simulink model "HW5"  (R2023b)
settings: Solver=FixedStepAuto  StartTime=0.0  StopTime=100  FixedStep=0.01  RelTol=1e-3
settings Model: Creator=ArshiaGosh  LastModifiedBy=ArshiaGosh

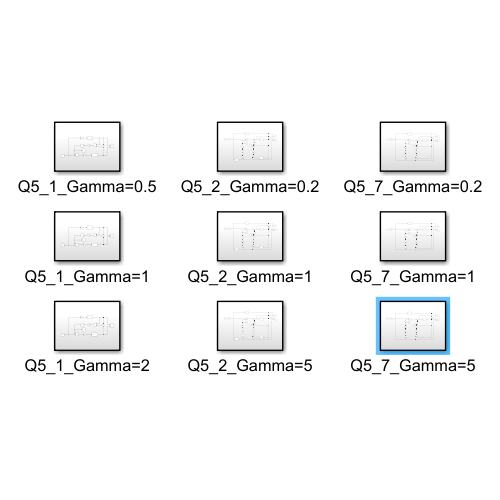
[thumbnail: Simulink's stored preview of the top-level diagram]
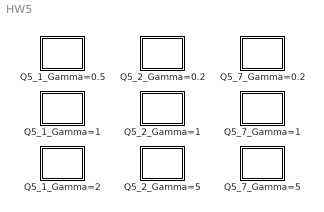
== system HW5 ==
  Q5_1_Gamma=0.5 : Subsystem
  Q5_1_Gamma=1 : Subsystem
  Q5_1_Gamma=2 : Subsystem
  Q5_2_Gamma=0.2 : Subsystem
  Q5_2_Gamma=1 : Subsystem
  Q5_2_Gamma=5 : Subsystem
  Q5_7_Gamma=0.2 : Subsystem
  Q5_7_Gamma=1 : Subsystem
  Q5_7_Gamma=5 : Subsystem

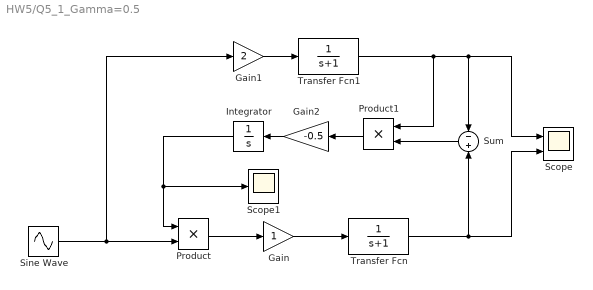
== system HW5/Q5_1_Gamma=0.5 ==
  Gain : Gain
  Gain1 : Gain  Gain=2
  Gain2 : Gain  Gain=-0.5
  Integrator : Integrator
  Product : Product
  Product1 : Product
  Scope : Scope  NumInputPorts=2
  Scope1 : Scope
  Sine Wave : Sin  SampleTime=0
  Sum : Sum  Inputs=-+
  Transfer Fcn : TransferFcn  Denominator=[1 1]
  Transfer Fcn1 : TransferFcn  Denominator=[1 1]
  wires:
  Product/1 -> Gain/1
  Gain/1 -> Transfer Fcn/1
  Transfer Fcn/1 -> Scope/2, Sum/2
  Gain1/1 -> Transfer Fcn1/1
  Transfer Fcn1/1 -> Scope/1, Sum/1, Product1/1
  Sum/1 -> Product1/2
  Gain2/1 -> Integrator/1
  Product1/1 -> Gain2/1
  Integrator/1 -> Scope1/1, Product/1
  Sine Wave/1 -> Gain1/1, Product/2

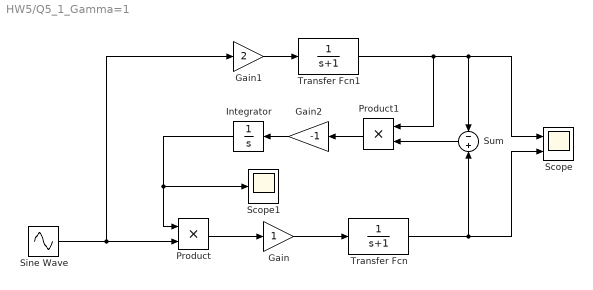
== system HW5/Q5_1_Gamma=1 ==
  Gain : Gain
  Gain1 : Gain  Gain=2
  Gain2 : Gain  Gain=-1
  Integrator : Integrator
  Product : Product
  Product1 : Product
  Scope : Scope  NumInputPorts=2
  Scope1 : Scope
  Sine Wave : Sin  SampleTime=0
  Sum : Sum  Inputs=-+
  Transfer Fcn : TransferFcn  Denominator=[1 1]
  Transfer Fcn1 : TransferFcn  Denominator=[1 1]
  wires:
  Sine Wave/1 -> Product/2, Gain1/1
  Integrator/1 -> Product/1, Scope1/1
  Product1/1 -> Gain2/1
  Gain2/1 -> Integrator/1
  Sum/1 -> Product1/2
  Transfer Fcn1/1 -> Product1/1, Sum/1, Scope/1
  Gain1/1 -> Transfer Fcn1/1
  Transfer Fcn/1 -> Sum/2, Scope/2
  Gain/1 -> Transfer Fcn/1
  Product/1 -> Gain/1

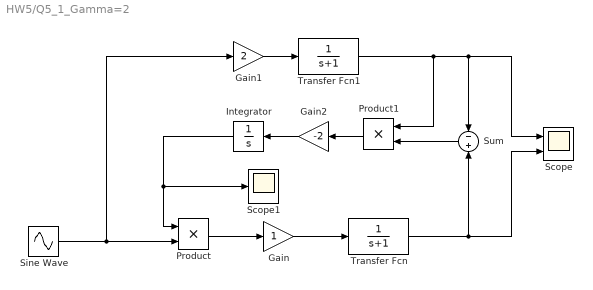
== system HW5/Q5_1_Gamma=2 ==
  Gain : Gain
  Gain1 : Gain  Gain=2
  Gain2 : Gain  Gain=-2
  Integrator : Integrator
  Product : Product
  Product1 : Product
  Scope : Scope  NumInputPorts=2
  Scope1 : Scope
  Sine Wave : Sin  SampleTime=0
  Sum : Sum  Inputs=-+
  Transfer Fcn : TransferFcn  Denominator=[1 1]
  Transfer Fcn1 : TransferFcn  Denominator=[1 1]
  wires:
  Product/1 -> Gain/1
  Gain/1 -> Transfer Fcn/1
  Transfer Fcn/1 -> Scope/2, Sum/2
  Gain1/1 -> Transfer Fcn1/1
  Transfer Fcn1/1 -> Scope/1, Sum/1, Product1/1
  Sum/1 -> Product1/2
  Gain2/1 -> Integrator/1
  Product1/1 -> Gain2/1
  Integrator/1 -> Scope1/1, Product/1
  Sine Wave/1 -> Gain1/1, Product/2

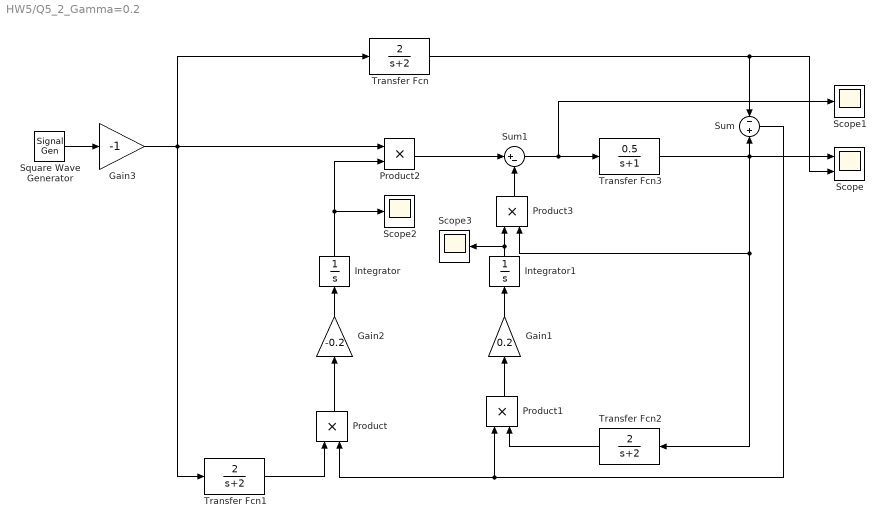
== system HW5/Q5_2_Gamma=0.2 ==
  Gain1 : Gain  Gain=0.2
  Gain2 : Gain  Gain=-0.2
  Gain3 : Gain  Gain=-1
  Integrator : Integrator
  Integrator1 : Integrator
  Product{,1..3} (4 alike) : Product
  Scope : Scope  NumInputPorts=2
  Scope1 : Scope
  Scope2 : Scope
  Scope3 : Scope
  Square Wave Generator : SignalGenerator  WaveForm=square  Frequency=0.30  Units=rad/sec
  Sum : Sum  Inputs=-+
  Sum1 : Sum  Inputs=|+-
  Transfer Fcn : TransferFcn  Numerator=[2]  Denominator=[1 2]
  Transfer Fcn1 : TransferFcn  Numerator=[2]  Denominator=[1 2]
  Transfer Fcn2 : TransferFcn  Numerator=[2]  Denominator=[1 2]
  Transfer Fcn3 : TransferFcn  Numerator=[0.5]  Denominator=[1 1]
  wires:
  Square Wave Generator/1 -> Gain3/1
  Transfer Fcn/1 -> Sum/1, Scope/2
  Transfer Fcn3/1 -> Product3/2, Transfer Fcn2/1, Sum/2, Scope/1
  Sum/1 -> Product1/1, Product/2
  Transfer Fcn1/1 -> Product/1
  Transfer Fcn2/1 -> Product1/2
  Gain2/1 -> Integrator/1
  Product/1 -> Gain2/1
  Integrator/1 -> Scope2/1, Product2/2
  Sum1/1 -> Scope1/1, Transfer Fcn3/1
  Product2/1 -> Sum1/1
  Product1/1 -> Gain1/1
  Gain1/1 -> Integrator1/1
  Product3/1 -> Sum1/2
  Gain3/1 -> Transfer Fcn/1, Product2/1, Transfer Fcn1/1
  Integrator1/1 -> Product3/1, Scope3/1

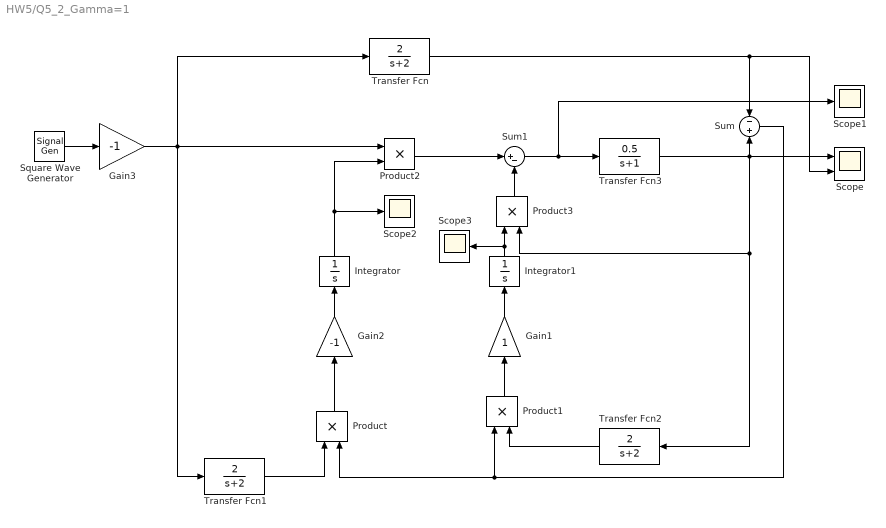
== system HW5/Q5_2_Gamma=1 ==
  Gain1 : Gain
  Gain2 : Gain  Gain=-1
  Gain3 : Gain  Gain=-1
  Integrator : Integrator
  Integrator1 : Integrator
  Product{,1..3} (4 alike) : Product
  Scope : Scope  NumInputPorts=2
  Scope1 : Scope
  Scope2 : Scope
  Scope3 : Scope
  Square Wave Generator : SignalGenerator  WaveForm=square  Frequency=0.30  Units=rad/sec
  Sum : Sum  Inputs=-+
  Sum1 : Sum  Inputs=|+-
  Transfer Fcn : TransferFcn  Numerator=[2]  Denominator=[1 2]
  Transfer Fcn1 : TransferFcn  Numerator=[2]  Denominator=[1 2]
  Transfer Fcn2 : TransferFcn  Numerator=[2]  Denominator=[1 2]
  Transfer Fcn3 : TransferFcn  Numerator=[0.5]  Denominator=[1 1]
  wires:
  Integrator1/1 -> Scope3/1, Product3/1
  Gain3/1 -> Transfer Fcn1/1, Product2/1, Transfer Fcn/1
  Product3/1 -> Sum1/2
  Gain1/1 -> Integrator1/1
  Product1/1 -> Gain1/1
  Product2/1 -> Sum1/1
  Sum1/1 -> Transfer Fcn3/1, Scope1/1
  Integrator/1 -> Product2/2, Scope2/1
  Product/1 -> Gain2/1
  Gain2/1 -> Integrator/1
  Transfer Fcn2/1 -> Product1/2
  Transfer Fcn1/1 -> Product/1
  Sum/1 -> Product/2, Product1/1
  Transfer Fcn3/1 -> Scope/1, Sum/2, Transfer Fcn2/1, Product3/2
  Transfer Fcn/1 -> Scope/2, Sum/1
  Square Wave Generator/1 -> Gain3/1

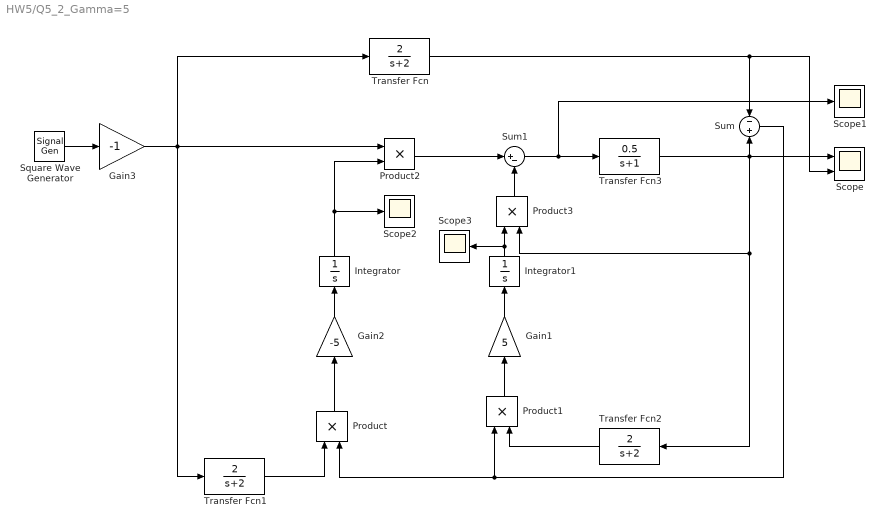
== system HW5/Q5_2_Gamma=5 ==
  Gain1 : Gain  Gain=5
  Gain2 : Gain  Gain=-5
  Gain3 : Gain  Gain=-1
  Integrator : Integrator
  Integrator1 : Integrator
  Product{,1..3} (4 alike) : Product
  Scope : Scope  NumInputPorts=2
  Scope1 : Scope
  Scope2 : Scope
  Scope3 : Scope
  Square Wave Generator : SignalGenerator  WaveForm=square  Frequency=0.30  Units=rad/sec
  Sum : Sum  Inputs=-+
  Sum1 : Sum  Inputs=|+-
  Transfer Fcn : TransferFcn  Numerator=[2]  Denominator=[1 2]
  Transfer Fcn1 : TransferFcn  Numerator=[2]  Denominator=[1 2]
  Transfer Fcn2 : TransferFcn  Numerator=[2]  Denominator=[1 2]
  Transfer Fcn3 : TransferFcn  Numerator=[0.5]  Denominator=[1 1]
  wires:
  Square Wave Generator/1 -> Gain3/1
  Transfer Fcn/1 -> Sum/1, Scope/2
  Transfer Fcn3/1 -> Product3/2, Transfer Fcn2/1, Sum/2, Scope/1
  Sum/1 -> Product1/1, Product/2
  Transfer Fcn1/1 -> Product/1
  Transfer Fcn2/1 -> Product1/2
  Gain2/1 -> Integrator/1
  Product/1 -> Gain2/1
  Integrator/1 -> Scope2/1, Product2/2
  Sum1/1 -> Scope1/1, Transfer Fcn3/1
  Product2/1 -> Sum1/1
  Product1/1 -> Gain1/1
  Gain1/1 -> Integrator1/1
  Product3/1 -> Sum1/2
  Gain3/1 -> Transfer Fcn/1, Product2/1, Transfer Fcn1/1
  Integrator1/1 -> Product3/1, Scope3/1

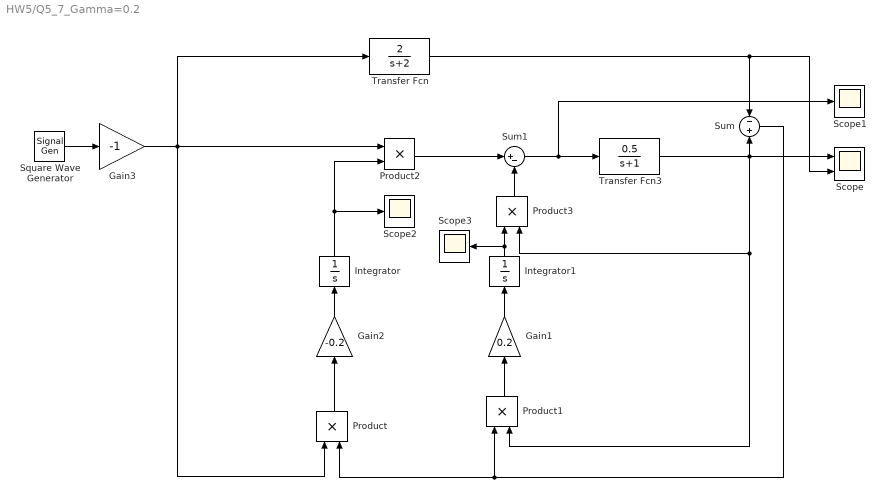
== system HW5/Q5_7_Gamma=0.2 ==
  Gain1 : Gain  Gain=0.2
  Gain2 : Gain  Gain=-0.2
  Gain3 : Gain  Gain=-1
  Integrator : Integrator
  Integrator1 : Integrator
  Product{,1..3} (4 alike) : Product
  Scope : Scope  NumInputPorts=2
  Scope1 : Scope
  Scope2 : Scope
  Scope3 : Scope
  Square Wave Generator : SignalGenerator  WaveForm=square  Frequency=0.30  Units=rad/sec
  Sum : Sum  Inputs=-+
  Sum1 : Sum  Inputs=|+-
  Transfer Fcn : TransferFcn  Numerator=[2]  Denominator=[1 2]
  Transfer Fcn3 : TransferFcn  Numerator=[0.5]  Denominator=[1 1]
  wires:
  Integrator1/1 -> Scope3/1, Product3/1
  Product3/1 -> Sum1/2
  Gain1/1 -> Integrator1/1
  Product1/1 -> Gain1/1
  Product2/1 -> Sum1/1
  Sum1/1 -> Transfer Fcn3/1, Scope1/1
  Integrator/1 -> Product2/2, Scope2/1
  Product/1 -> Gain2/1
  Gain2/1 -> Integrator/1
  Transfer Fcn3/1 -> Scope/1, Sum/2, Product1/2, Product3/2
  Gain3/1 -> Product/1, Product2/1, Transfer Fcn/1
  Sum/1 -> Product/2, Product1/1
  Transfer Fcn/1 -> Scope/2, Sum/1
  Square Wave Generator/1 -> Gain3/1

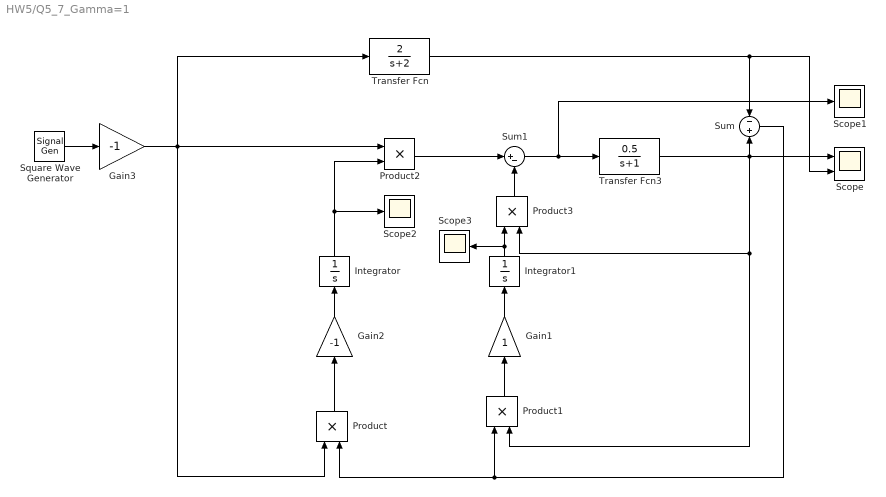
== system HW5/Q5_7_Gamma=1 ==
  Gain1 : Gain
  Gain2 : Gain  Gain=-1
  Gain3 : Gain  Gain=-1
  Integrator : Integrator
  Integrator1 : Integrator
  Product{,1..3} (4 alike) : Product
  Scope : Scope  NumInputPorts=2
  Scope1 : Scope
  Scope2 : Scope
  Scope3 : Scope
  Square Wave Generator : SignalGenerator  WaveForm=square  Frequency=0.30  Units=rad/sec
  Sum : Sum  Inputs=-+
  Sum1 : Sum  Inputs=|+-
  Transfer Fcn : TransferFcn  Numerator=[2]  Denominator=[1 2]
  Transfer Fcn3 : TransferFcn  Numerator=[0.5]  Denominator=[1 1]
  wires:
  Square Wave Generator/1 -> Gain3/1
  Transfer Fcn/1 -> Sum/1, Scope/2
  Sum/1 -> Product1/1, Product/2
  Gain3/1 -> Transfer Fcn/1, Product2/1, Product/1
  Transfer Fcn3/1 -> Product3/2, Product1/2, Sum/2, Scope/1
  Gain2/1 -> Integrator/1
  Product/1 -> Gain2/1
  Integrator/1 -> Scope2/1, Product2/2
  Sum1/1 -> Scope1/1, Transfer Fcn3/1
  Product2/1 -> Sum1/1
  Product1/1 -> Gain1/1
  Gain1/1 -> Integrator1/1
  Product3/1 -> Sum1/2
  Integrator1/1 -> Product3/1, Scope3/1

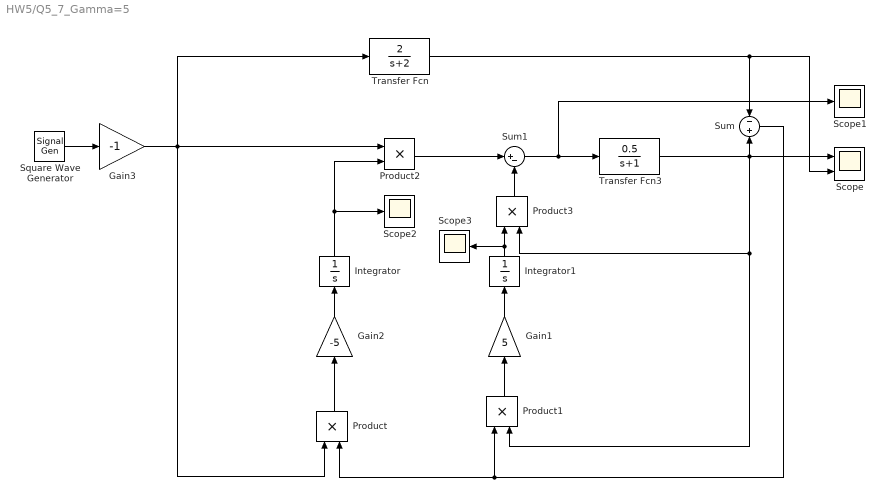
== system HW5/Q5_7_Gamma=5 ==
  Gain1 : Gain  Gain=5
  Gain2 : Gain  Gain=-5
  Gain3 : Gain  Gain=-1
  Integrator : Integrator
  Integrator1 : Integrator
  Product{,1..3} (4 alike) : Product
  Scope : Scope  NumInputPorts=2
  Scope1 : Scope
  Scope2 : Scope
  Scope3 : Scope
  Square Wave Generator : SignalGenerator  WaveForm=square  Frequency=0.30  Units=rad/sec
  Sum : Sum  Inputs=-+
  Sum1 : Sum  Inputs=|+-
  Transfer Fcn : TransferFcn  Numerator=[2]  Denominator=[1 2]
  Transfer Fcn3 : TransferFcn  Numerator=[0.5]  Denominator=[1 1]
  wires:
  Integrator1/1 -> Scope3/1, Product3/1
  Product3/1 -> Sum1/2
  Gain1/1 -> Integrator1/1
  Product1/1 -> Gain1/1
  Product2/1 -> Sum1/1
  Sum1/1 -> Transfer Fcn3/1, Scope1/1
  Integrator/1 -> Product2/2, Scope2/1
  Product/1 -> Gain2/1
  Gain2/1 -> Integrator/1
  Transfer Fcn3/1 -> Scope/1, Sum/2, Product1/2, Product3/2
  Gain3/1 -> Product/1, Product2/1, Transfer Fcn/1
  Sum/1 -> Product/2, Product1/1
  Transfer Fcn/1 -> Scope/2, Sum/1
  Square Wave Generator/1 -> Gain3/1
